simulink model "Ohm_Law"  (R2024b)
settings: Solver=VariableStepAuto  StartTime=0.0  StopTime=5  MaxStep=1e-4  RelTol=1e-3
libraries: fl_lib x10, nesl_utility x8, simulink x2
settings Model: Creator=Hp  LastModifiedBy=Hp

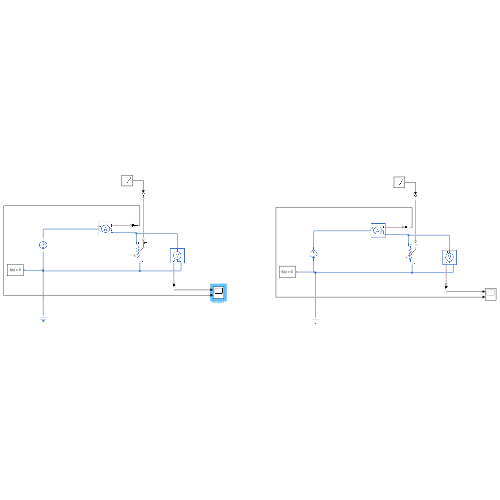
[thumbnail: Simulink's stored preview of the top-level diagram]
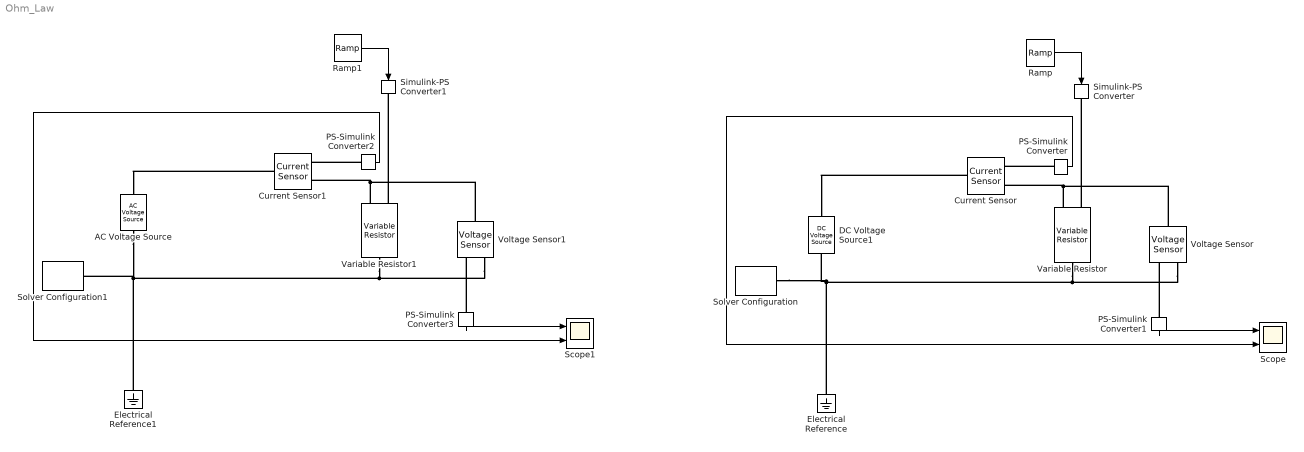
== system Ohm_Law ==
  AC Voltage Source : fl_lib/Electrical/Electrical Sources/AC Voltage Source  amp=50 V  shift=0 deg  frequency=50 Hz
  Current Sensor : fl_lib/Electrical/Electrical Sensors/Current Sensor
  Current Sensor1 : fl_lib/Electrical/Electrical Sensors/Current Sensor
  DC Voltage Source1 : fl_lib/Electrical/Electrical Sources/DC Voltage Source  v0=12 V
  Electrical Reference : fl_lib/Electrical/Electrical Elements/Electrical Reference
  Electrical Reference1 : fl_lib/Electrical/Electrical Elements/Electrical Reference
  PS-Simulink Converter{,1..3} (4 alike) : nesl_utility/PS-Simulink Converter  PhysicalDomain=network_engine_domain  SubClassName=ps_output  LeftPortType=input  RightPortType=output  PseudoPeriodic=off  Frequencies=[]  VectorFormat=inherit  Unit=inherit  AffineConversion=off
  Ramp : simulink/Sources/Ramp  slope=5  start=0  InitialOutput=0
  Ramp1 : simulink/Sources/Ramp  slope=5  start=0  InitialOutput=0
  Scope : Scope  NumInputPorts=2
  Scope1 : Scope  NumInputPorts=2
  Simulink-PS Converter : nesl_utility/Simulink-PS Converter  PhysicalDomain=network_engine_domain  SubClassName=ps_input  LeftPortType=input  RightPortType=output  PseudoPeriodic=off  Frequencies=[]  NoiseDistribution=none  NoiseParameters=[]  Unit=1  AffineConversion=off  FilteringAndDerivatives=provide  SimscapeFilterOrder=1  InputFilterTimeConstant=0.001  UdotUserProvided=0
  Simulink-PS Converter1 : nesl_utility/Simulink-PS Converter  PhysicalDomain=network_engine_domain  SubClassName=ps_input  LeftPortType=input  RightPortType=output  PseudoPeriodic=off  Frequencies=[]  NoiseDistribution=none  NoiseParameters=[]  Unit=1  AffineConversion=off  FilteringAndDerivatives=provide  SimscapeFilterOrder=1  InputFilterTimeConstant=0.001  UdotUserProvided=0
  Solver Configuration : nesl_utility/Solver Configuration  PhysicalDomain=network_engine_domain  SubClassName=solver  LeftPortType=input  RightPortType=generic  Tones=[]  Harmonics=[]  SimulateNoise=off  Profile=off  UseLocalSampling=off  EnableSwitchedLinearOptims=on  FrequencyDomain=off  UseCCode=off  RelTol=0.001  AbsTol=0.001  MinStep=1e-09  ToWorkspace=off  RevertToSquareIcSolve=off  NumHomotopyIterations=100  PhasorMode=off  PhasorModeNumHarmonics=1  ConsistencySolver=NEWTON_XTOL_AFTER_FTOL  IndexReductionMethod=DerivativeReplacement  DoDC=off  ResidualTolerance=1e-09  ConsistencyTolSource=GLOBAL  ConsistencyAbsTol=0.001  ConsistencyRelTol=0.001  ConsistencyTolFactor=0.001  UseLocalSolver=off  LocalSolverChoice=NE_BACKWARD_EULER_ADVANCER  ResolveIndetEquations=on  FunctionEvalNumThread=1  LocalSolverSampleTime=0.001  DoFixedCost=off  MaxNonlinIter=3  MaxModeIter=2  ComputeImpulses=off  ImpulseIterations=2  LinearAlgebra=auto  LinearAlgebraNumThread=0  EquationFormulation=NE_TIME_EF  DelaysMemoryBudget=1024  AutomaticFiltering=on  FilteringTimeConstant=0.001  PartitionStorageMethod=AS_NEEDED  PartitionMemoryBudget=1024  PartitionMethod=ROBUST  MultibodyUseLocalSolver=off  MultibodyLocalSolverChoice=ODE1  MultibodyLocalSolverSampleTime=0.001
  Solver Configuration1 : nesl_utility/Solver Configuration  PhysicalDomain=network_engine_domain  SubClassName=solver  LeftPortType=input  RightPortType=generic  Tones=[]  Harmonics=[]  SimulateNoise=off  Profile=off  UseLocalSampling=off  EnableSwitchedLinearOptims=on  FrequencyDomain=off  UseCCode=off  RelTol=0.001  AbsTol=0.001  MinStep=1e-09  ToWorkspace=off  RevertToSquareIcSolve=off  NumHomotopyIterations=100  PhasorMode=off  PhasorModeNumHarmonics=1  ConsistencySolver=NEWTON_XTOL_AFTER_FTOL  IndexReductionMethod=DerivativeReplacement  DoDC=off  ResidualTolerance=1e-09  ConsistencyTolSource=GLOBAL  ConsistencyAbsTol=0.001  ConsistencyRelTol=0.001  ConsistencyTolFactor=0.001  UseLocalSolver=off  LocalSolverChoice=NE_BACKWARD_EULER_ADVANCER  ResolveIndetEquations=on  FunctionEvalNumThread=1  LocalSolverSampleTime=0.001  DoFixedCost=off  MaxNonlinIter=3  MaxModeIter=2  ComputeImpulses=off  ImpulseIterations=2  LinearAlgebra=auto  LinearAlgebraNumThread=0  EquationFormulation=NE_TIME_EF  DelaysMemoryBudget=1024  AutomaticFiltering=on  FilteringTimeConstant=0.001  PartitionStorageMethod=AS_NEEDED  PartitionMemoryBudget=1024  PartitionMethod=ROBUST  MultibodyUseLocalSolver=off  MultibodyLocalSolverChoice=ODE1  MultibodyLocalSolverSampleTime=0.001
  Variable Resistor : fl_lib/Electrical/Electrical Elements/Variable Resistor  Rmin=5 Ohm  thermalEnable=false  thermal_mass=1 J/K  i_specify=off  i_priority=None  i=0 A  i_nominal_specify=off  i_nominal_value=1  i_nominal_unit=A  v_specify=off  v_priority=None  v=0 V  v_nominal_specify=off  v_nominal_value=1  v_nominal_unit=V  T_specify=off  T_priority=None  T=300 K  T_nominal_specify=off  T_nominal_value=1  T_nominal_unit=K
  Variable Resistor1 : fl_lib/Electrical/Electrical Elements/Variable Resistor  Rmin=5 Ohm  thermalEnable=false  thermal_mass=1 J/K  i_specify=off  i_priority=None  i=0 A  i_nominal_specify=off  i_nominal_value=1  i_nominal_unit=A  v_specify=off  v_priority=None  v=0 V  v_nominal_specify=off  v_nominal_value=1  v_nominal_unit=V  T_specify=off  T_priority=None  T=300 K  T_nominal_specify=off  T_nominal_value=1  T_nominal_unit=K
  Voltage Sensor : fl_lib/Electrical/Electrical Sensors/Voltage Sensor
  Voltage Sensor1 : fl_lib/Electrical/Electrical Sensors/Voltage Sensor
  wires:
  Ramp/1 -> Simulink-PS Converter/1
  PS-Simulink Converter1/1 -> Scope/1
  PS-Simulink Converter/1 -> Scope/2
  PS-Simulink Converter2/1 -> Scope1/2
  Ramp1/1 -> Simulink-PS Converter1/1
  PS-Simulink Converter3/1 -> Scope1/1
  connections:
  Current Sensor/LConn1 -- DC Voltage Source1/LConn1
  Variable Resistor/LConn2 -- Voltage Sensor/LConn1 -- Current Sensor/RConn2
  Variable Resistor/RConn1 -- Voltage Sensor/RConn2 -- Solver Configuration/RConn1 -- DC Voltage Source1/RConn1 -- Electrical Reference/LConn1
  PS-Simulink Converter/LConn1 -- Current Sensor/RConn1
  Variable Resistor/LConn1 -- Simulink-PS Converter/RConn1
  PS-Simulink Converter1/LConn1 -- Voltage Sensor/RConn1
  Variable Resistor1/RConn1 -- Voltage Sensor1/RConn2 -- AC Voltage Source/RConn1 -- Solver Configuration1/RConn1 -- Electrical Reference1/LConn1
  Variable Resistor1/LConn2 -- Voltage Sensor1/LConn1 -- Current Sensor1/RConn2
  PS-Simulink Converter3/LConn1 -- Voltage Sensor1/RConn1
  PS-Simulink Converter2/LConn1 -- Current Sensor1/RConn1
  Variable Resistor1/LConn1 -- Simulink-PS Converter1/RConn1
  Current Sensor1/LConn1 -- AC Voltage Source/LConn1
